simulink model "E3_"  (R2024a)
settings: Solver=VariableStepAuto  StartTime=0.0  StopTime=10.0  RelTol=1e-3
settings Model: Creator=Sanagostar  LastModifiedBy=Sanagostar

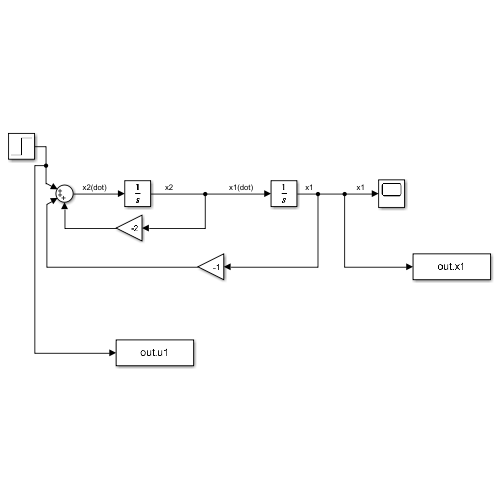
[thumbnail: Simulink's stored preview of the top-level diagram]
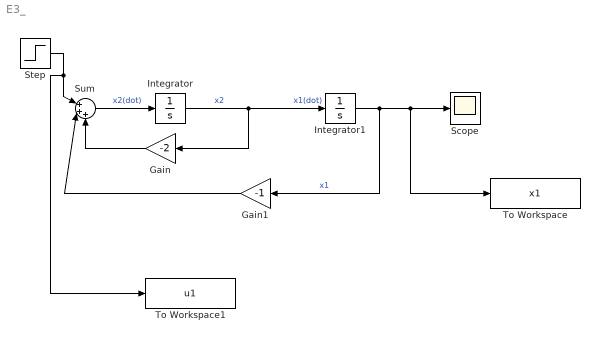
== system E3_ ==
  Gain : Gain  Gain=-2
  Gain1 : Gain  Gain=-1
  Integrator : Integrator
  Integrator1 : Integrator
  Scope : Scope
  Step : Step  Time=0  SampleTime=0
  Sum : Sum  Inputs=|+++
  To Workspace : ToWorkspace  VariableName=x1  SaveFormat=Timeseries  SampleTime=-1
  To Workspace1 : ToWorkspace  VariableName=u1  SaveFormat=Timeseries  SampleTime=-1
  wires:
  Integrator/1 -> Gain/1, Integrator1/1  "x2                          x1(dot)"
  Sum/1 -> Integrator/1  "x2(dot)"
  Gain1/1 -> Sum/2
  Gain/1 -> Sum/3
  Integrator1/1 -> To Workspace/1, Scope/1, Gain1/1  "x1"
  Step/1 -> To Workspace1/1, Sum/1
